simulink model "Lab6"  (R2023a)
settings: Solver=FixedStepDiscrete  StartTime=0.0  StopTime=1000  FixedStep=1/MultiDeviceDAQ_getSampleRate  RelTol=1e-3  EnableMultiTasking=on
InitFcn:
  | clear global handle
  | 
  | clear global userData
  | 
  | tmp_string = gcb;
  | modelname = tmp_string(1:findstr(tmp_string, '/'));
  | method_name = sprintf('%sSignal Processing', modelname);
  | method_val = get_param(method_name,'method');
  | 
  | if exist('P300classifier') ~=1 || (strcmp(method_val, 'Linear Discriminant Analysis') && P300classifier.method ~= 1) || (strcmp(method_val, 'Support Vector Machine') && P300classifier.method ~= 2)
  | try
  | if strcmp(method_val, 'Linear Discriminant Analysis')
  | load lda_rowcolumn_classifier.mat
  | elseif strcmp(method_val, 'Support Vector Machine')
  | load svm_rowcolumn_classifier.mat
  | else
  | global P300classifier
  | P300classifier.method = 0;
  | end
  | catch
  | global P300classifier
  | P300classifier.method = 0;
  | end
  | end
StartFcn:
  | tmp_string = gcb;
  | modelname = tmp_string(1:findstr(tmp_string, '/'));
  | stopsimu_name = sprintf('%sRowCol Character Speller/StopSimu', modelname);
  | set_param(stopsimu_name,'Gain','0');
undefined symbols (not defined in the file): MultiDeviceDAQ_getNumChannels, MultiDeviceDAQ_getSampleRate
libraries: FeatureExtraction x2, Transformation x2, Visualization x2, dspstat3 x1, Preprocessing x1, simulink x1, Classification x1, DataAcquisition x1
settings Model: ModifiedByFormat=g.tec  Creator=circuit  LastModifiedBy=g.tec
settings SolverCC: AlgebraicLoopSolver=TrustRegion
settings DataIOCC: LimitDataPoints=on  SaveFormat=Array  SignalLoggingSaveFormat=ModelDataLogs  ReturnWorkspaceOutputs=off
settings OptimizationCC: ExpressionDepthLimit=2147483647  InitFltsAndDblsToZero=on  LifeSpan=inf
settings DebuggingCC: SaveWithParameterizedLinksMsg=none  UnderspecifiedInitializationDetection=Classic  MergeDetectMultiDrivingBlocksExec=none  SignalResolutionControl=TryResolveAllWithWarning  SolverPrmCheckMsg=warning  MultiTaskDSMMsg=warning  MultiTaskCondExecSysMsg=none  FcnCallInpInsideContextMsg=warning  UnconnectedInputMsg=warning  UnconnectedOutputMsg=warning  UnconnectedLineMsg=warning  FrameProcessingCompatibilityMsg=none  StateNameClashWarn=warning  SFUnexpectedBacktrackingDiag=warning  SFNoUnconditionalDefaultTransitionDiag=warning  SFExecutionAtInitializationDiag=none  ArithmeticOperatorsInVariantConditions=warning
settings HardwareCC: ProdBitPerPointer=32  ProdBitPerSizeT=32  ProdBitPerPtrDiffT=32  ProdLargestAtomicFloat=None  ProdIntDivRoundTo=Undefined  ProdEndianess=Unspecified  ProdWordSize=32  ProdHWDeviceType=32-bit Generic
settings ModelReferenceCC: EnableRefExpFcnMdlSchedulingChecks=on  PropagateSignalLabelsOutOfModel=off
settings SFSimCC: SimUseLocalCustomCode=off  CustomCodeUndefinedFunction=UseInterfaceOnly
settings RTWCC: RTWUseLocalCustomCode=off
settings CodeAppCC: StateflowObjectComments=on
settings GRTTargetCC: TargetFcnLib=ansi_tfl_tmw.mat  TargetLangStandard=C89/C90 (ANSI)  CombineOutputUpdateFcns=off  GRTInterface=on
settings ConfigComp: CovMetricSettings=dw  CovSaveCumulativeToWorkspaceVar=on  CovSaveSingleToWorkspaceVar=on  CovExternalEMLEnable=off

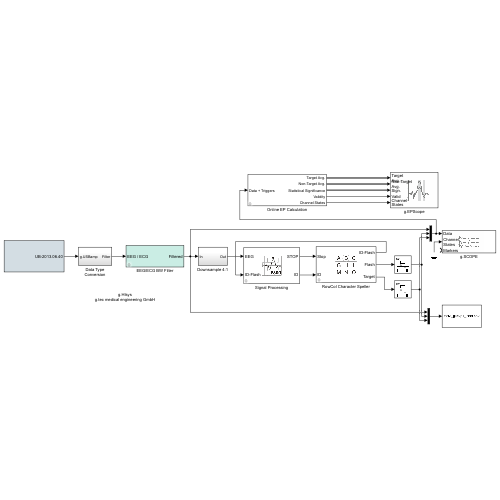
[thumbnail: Simulink's stored preview of the top-level diagram]
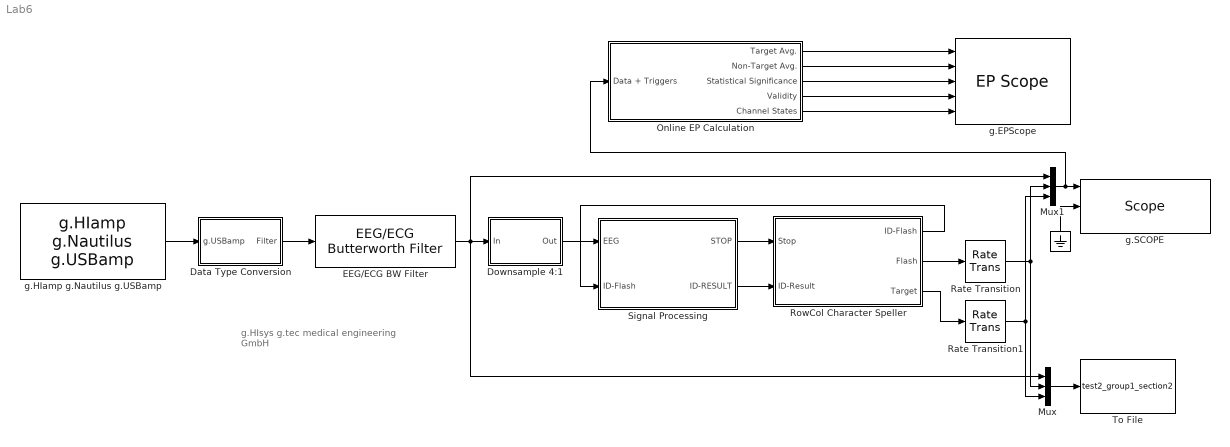
== system Lab6 ==
  note: g.HIsys
      | g.tec medical engineering GmbH
  " " : Ground
  Data Type Conversion : Subsystem
  Downsample 4:1 : Subsystem
  EEG/ECG BW Filter : Preprocessing/EEG//ECG Butterworth Filter  Order=6  LowerFreq=0.1  UpperFreq=30  SampFreq=MultiDeviceDAQ_getSampleRate
      settings: SourceProductName=g.HIsys
  Mux : Mux  Inputs=3
  Mux1 : Mux  Inputs=3
  Online EP Calculation : Subsystem  mask(Online EP Calculation){data_ch_count=MultiDeviceDAQ_getNumChannels, sampletime=1/MultiDeviceDAQ_getSampleRate}
      mask prompts: data_ch_count "Number of data channels:"; sampletime "Sampling time"
      mask help:
      | Calculates the target and non-target average of the incoming data and performs statistical significance analysis of target and non-target frames.
      | The data coming in must contain 'Number of data channel' data channels, trigger IDs and target triggers.
  Rate Transition : RateTransition
  Rate Transition1 : RateTransition
  RowCol Character Speller : Subsystem  mask(Single Character Flash Speller){mode=Copy Spelling, flashtime=100, darktime=75}
      mask prompts: flashtime "Flash time [ms]:"; darktime "Dark time [ms]:"
      mask help: Displays a 36 character matrix. A row or a column of characters is flashing up for a specific time in a random and sequential order. The dark time is the time between the characters.
      mask Help:
      | Displays a 36 character matrix. A row or a column of characters is flashing up for a specific time in a random and sequential order. The dark time is the time between the characters. If the row/column is flashing up the ID-Flash is transmitted for the Signal Processing. Flash contains the ID of every character in the row/column. Target is one if a specific character for the copy spelling mode flashes up. <br><br>
      | 
      | Mode - can be Copy Spelling or Free Spelling<br><br>
      | Flash time [ms] - time that character is shown on screen <br><br>
      | Dark time [ms] - time between the characters
      mask TypeOptions mode: Copy Spelling | Free Spelling
      mask Display:
      | image(imread('speller2.tif'))
      | port_label('output',1,'ID-Flash')
      | port_label('output',2,'Flash')
      | port_label('output',3,'Target')
      | port_label('input',1,'Stop')
      | port_label('input',2,'ID')
  Signal Processing : Subsystem  mask(P300 Signal Processing){windTime=800, runmax=15, channels=8, method=Linear Discriminant Analysis}
      mask prompts: windTime "Buffer length [ms]:"; runmax "Number of flashes:"; channels "Number of channels:"; method "Classification Method:"
      mask help: The block buffers EEG data for each ID-Flash obtained. As soon as M (Number of flashes) characters of each ID are obtained a STOP command is sent and the maximum P300 is calculated and applied on output ID.
      mask Help:
      | P300 Signal Processing block. The block buffers EEG data for each ID-Flash obtained. As soon as M (Number of flashes) characters of each ID are obtained a STOP command is sent. Then the maximum P300 is calculated and the character ID is sent. <br><br>
      | 
      | Buffer length [ms] - enter the EEG data buffer size <br><br>
      | Number of flashes - enter the number each character should flash up <br><br>
      mask TypeOptions method: Linear Discriminant Analysis | Support Vector Machine
      mask Display:
      | image(imread('p3002.tif'))
      | port_label('output', 1, 'STOP')
      | port_label('output', 2, 'ID')
      | port_label('input', 1, 'EEG')
      | port_label('input', 2, 'ID-Flash')
  To File : ToFile  Filename=test2_group1_section2  MatrixName=y  SampleTime=1/MultiDeviceDAQ_getSampleRate
  g.EPScope : Visualization/EP Scope
      settings: SourceProductName=g.HIsys
  g.HIamp g.Nautilus g.USBamp : DataAcquisition/g.HIamp g.Nautilus g.USBamp  cfgUpdated=739906.4436  numDevices=2  deviceSR=[500 250 ]  deviceChannels=[9 4 ]  numSR=[2 ]  SRIndexPerDevice=[1 0 ]
      settings: SourceProductName=g.HIsys
  g.SCOPE : Visualization/Scope
      settings: SourceProductName=g.HIsys
  wires:
  g.HIamp g.Nautilus g.USBamp/1 -> Data Type Conversion/1(g.USBamp)
  Data Type Conversion/1(Filter) -> EEG/ECG BW Filter/1
  EEG/ECG BW Filter/1 -> Mux1/1, Downsample 4:1/1(In), Mux/1
  Signal Processing/1(STOP) -> RowCol Character Speller/1(Stop)
  Signal Processing/2(ID-RESULT) -> RowCol Character Speller/2(ID-Result)
  RowCol Character Speller/1(ID-Flash) -> Signal Processing/2(ID-Flash)
  RowCol Character Speller/2(Flash) -> Rate Transition/1
  RowCol Character Speller/3(Target) -> Rate Transition1/1
  Rate Transition/1 -> Mux1/2, Mux/2
  Rate Transition1/1 -> Mux1/3, Mux/3
  Downsample 4:1/1(Out) -> Signal Processing/1(EEG)
  Mux1/1 -> Online EP Calculation/1(Data + Triggers), g.SCOPE/1
  Mux/1 -> To File/1
  " "/1 -> g.SCOPE/2
  Online EP Calculation/2(Non-Target Avg.) -> g.EPScope/2
  Online EP Calculation/3(Statistical Significance) -> g.EPScope/3
  Online EP Calculation/4(Validity) -> g.EPScope/4
  Online EP Calculation/1(Target Avg.) -> g.EPScope/1
  Online EP Calculation/5(Channel States) -> g.EPScope/5

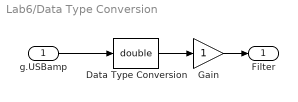
== system Lab6/Data Type Conversion ==
  g.USBamp : Inport  Priority=1
  Data Type Conversion : DataTypeConversion  OutDataTypeStr=double  SaturateOnIntegerOverflow=off  RndMeth=Floor
  Gain : Gain  SaturateOnIntegerOverflow=on  SampleTime=1/MultiDeviceDAQ_getSampleRate  OutDataTypeStr=Inherit: Same as input  ParamDataTypeStr=Inherit: Same as input
  Filter : Outport
  wires:
  Data Type Conversion/1 -> Gain/1
  g.USBamp/1 -> Data Type Conversion/1
  Gain/1 -> Filter/1

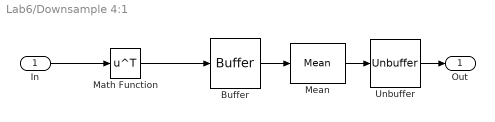
== system Lab6/Downsample 4:1 ==
  In : Inport
  Buffer : Buffer  N=4
  Math Function : Math  Operator=transpose  SignedPower=on
  Mean : dspstat3/Mean  run=off  InputProcessing=Columns as channels (frame based)  reset_popup=None  directionMode=Each column  dimension=1  roiEnable=off  roiType=Rectangles  roiPortion=Entire ROI  roiOutput=Individual statistics for each ROI  roiFlag=off  roundingMode=Floor  overflowMode=off  outputDataTypeStr=Inherit: Same as accumulator  outputMin=[]  outputMax=[]  outputLastDataTypeStr=Inherit: Same as accumulator
  Unbuffer : Unbuffer
  Out : Outport
  wires:
  Buffer/1 -> Mean/1
  Mean/1 -> Unbuffer/1
  In/1 -> Math Function/1
  Unbuffer/1 -> Out/1
  Math Function/1 -> Buffer/1

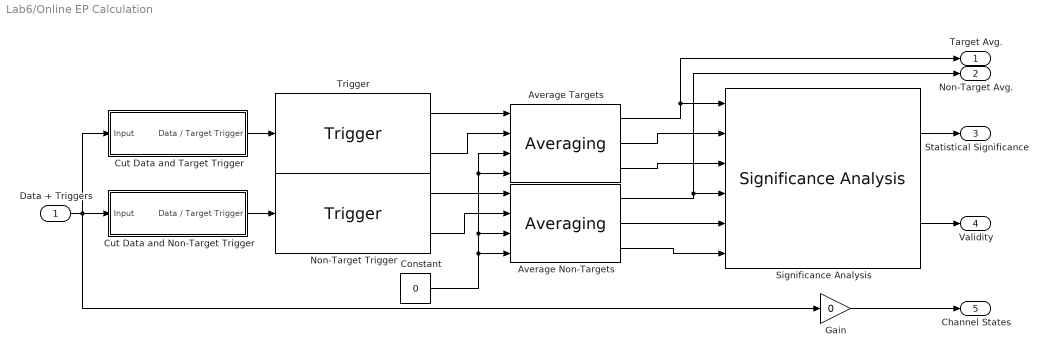
== system Lab6/Online EP Calculation ==
  Data + Triggers : Inport
  Average Non-Targets : FeatureExtraction/Averaging  mode_select=1 - average all data  mode=0  window=3  add_std=on  do_baseline_correction=off  baseline_interval=[0 0]  sampletime=sampletime
      settings: SourceProductName=g.HIsys
  Average Targets : FeatureExtraction/Averaging  mode_select=1 - average all data  mode=0  window=3  add_std=on  do_baseline_correction=off  baseline_interval=[0 0]  sampletime=sampletime
      settings: SourceProductName=g.HIsys
  Constant : Constant  Value=0
  Cut Data and Non-Target Trigger : Subsystem
  Cut Data and Target Trigger : Subsystem
  Gain : Gain  Gain=0
  Non-Target Trigger : Transformation/Trigger  trigchan=9  edge_select=RISING  edge=0  treshold=1  ext_treshold=off  windowsize=0.7  pretrigger=-0.1  sampletime=sampletime  validity_select=STANDARD (global validity flag for all channels)  validity=0  discardTriggerChannels=off
      settings: SourceProductName=g.HIsys
  Significance Analysis : Classification/Significance Analysis  sampletime=sampletime  pValue_select=4 - 0.95  pValue=3  update_mode_select=1 - any Group  update_mode=0
      settings: SourceProductName=g.HIsys
  Trigger : Transformation/Trigger  trigchan=9  edge_select=RISING  edge=0  treshold=1  ext_treshold=off  windowsize=0.7  pretrigger=-0.1  sampletime=sampletime  validity_select=STANDARD (global validity flag for all channels)  validity=0  discardTriggerChannels=off
      settings: SourceProductName=g.HIsys
  Target Avg. : Outport
  Non-Target Avg. : Outport  Port=2
  Statistical Significance : Outport  Port=3
  Validity : Outport  Port=4
  Channel States : Outport  Port=5
  wires:
  Data + Triggers/1 -> Cut Data and Target Trigger/1(Input), Cut Data and Non-Target Trigger/1(Input), Gain/1
  Average Targets/3 -> Significance Analysis/3
  Average Targets/2 -> Significance Analysis/2
  Average Non-Targets/2 -> Significance Analysis/5
  Average Non-Targets/3 -> Significance Analysis/6
  Significance Analysis/2 -> Validity/1
  Trigger/2 -> Average Targets/2
  Trigger/1 -> Average Targets/1
  Non-Target Trigger/1 -> Average Non-Targets/1
  Non-Target Trigger/2 -> Average Non-Targets/2
  Average Targets/1 -> Target Avg./1, Significance Analysis/1
  Average Non-Targets/1 -> Non-Target Avg./1, Significance Analysis/4
  Significance Analysis/1 -> Statistical Significance/1
  Gain/1 -> Channel States/1
  Cut Data and Target Trigger/1(Data / Target Trigger) -> Trigger/1
  Cut Data and Non-Target Trigger/1(Data / Target Trigger) -> Non-Target Trigger/1
  Constant/1 -> Average Non-Targets/4, Average Non-Targets/3, Average Targets/4, Average Targets/3

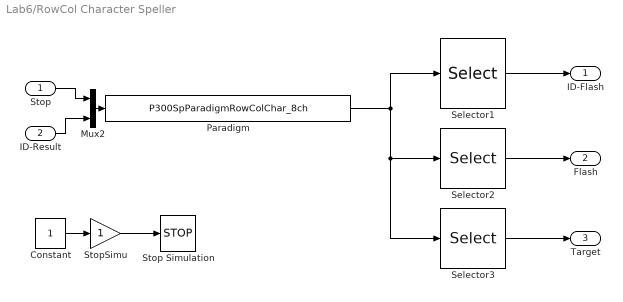
== system Lab6/RowCol Character Speller ==
  Stop : Inport
  ID-Result : Inport  Port=2
  Constant : Constant
  Mux2 : Mux  Inputs=2
  Paradigm : S-Function  FunctionName=P300SpParadigmRowColChar_8ch  Parameters=mode,flashtime,darktime,MultiDeviceDAQ_getSampleRate  SFunctionDeploymentMode=off  EnableBusSupport=off
  Selector1 : Selector  InputPortWidth=9  IndexOptions=Index vector (dialog)  Indices=1:7  OutputSizes=1
  Selector2 : Selector  InputPortWidth=9  IndexOptions=Index vector (dialog)  Indices=[8]  OutputSizes=1
  Selector3 : Selector  InputPortWidth=9  IndexOptions=Index vector (dialog)  Indices=[9]  OutputSizes=1
  Stop Simulation : Stop
  StopSimu : Gain
  ID-Flash : Outport
  Flash : Outport  Port=2
  Target : Outport  Port=3
  wires:
  Stop/1 -> Mux2/1
  ID-Result/1 -> Mux2/2
  Mux2/1 -> Paradigm/1
  Constant/1 -> StopSimu/1
  StopSimu/1 -> Stop Simulation/1
  Paradigm/1 -> Selector1/1, Selector2/1, Selector3/1
  Selector1/1 -> ID-Flash/1
  Selector2/1 -> Flash/1
  Selector3/1 -> Target/1

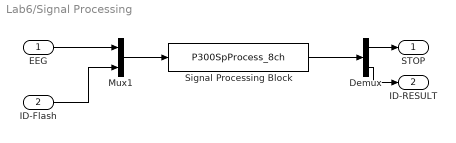
== system Lab6/Signal Processing ==
  EEG : Inport
  ID-Flash : Inport  Port=2
  Demux : Demux  Outputs=2
  Mux1 : Mux  Inputs=2
  Signal Processing Block : S-Function  FunctionName=P300SpProcess_8ch  Parameters=windTime, runmax, channels, method, P300classifier  SFunctionDeploymentMode=off  EnableBusSupport=off
  STOP : Outport
  ID-RESULT : Outport  Port=2
  wires:
  ID-Flash/1 -> Mux1/2
  Demux/1 -> STOP/1
  Demux/2 -> ID-RESULT/1
  Mux1/1 -> Signal Processing Block/1
  Signal Processing Block/1 -> Demux/1
  EEG/1 -> Mux1/1

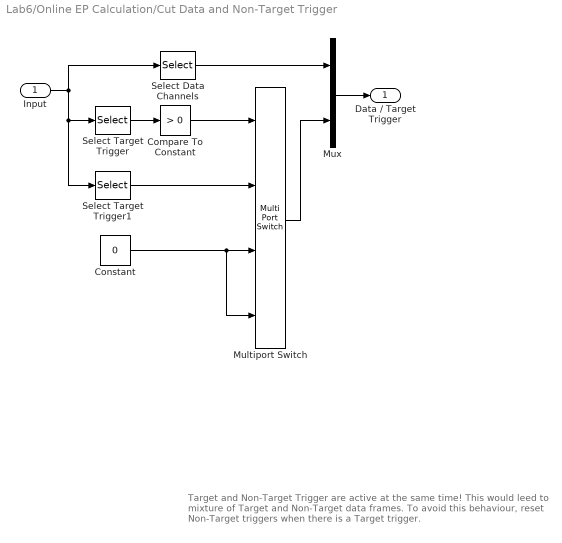
== system Lab6/Online EP Calculation/Cut Data and Non-Target Trigger ==
  note: Target and Non-Target Trigger are active at the same time!
      | This would leed to mixture of Target and Non-Target data frames.
      | To avoid this behaviour, reset Non-Target triggers when there is a Target trigger.
  Input : Inport
  Compare To Constant : simulink/Logic and Bit Operations/Compare To Constant  relop=>  const=0  OutDataTypeStr=uint8
  Constant : Constant  Value=0
  Multiport Switch : MultiPortSwitch  DataPortOrder=Zero-based contiguous  zeroidx=on  SaturateOnIntegerOverflow=off  InputSameDT=off
  Mux : Mux  Inputs=2
  Select Data Channels : Selector  InputPortWidth=data_ch_count + 2  IndexOptions=Index vector (dialog)  Indices=[1:data_ch_count]  OutputSizes=1
  Select Target Trigger : Selector  InputPortWidth=data_ch_count + 2  IndexOptions=Index vector (dialog)  Indices=data_ch_count+2  OutputSizes=1
  Select Target Trigger1 : Selector  InputPortWidth=data_ch_count + 2  IndexOptions=Index vector (dialog)  Indices=data_ch_count+1  OutputSizes=1
  Data / Target Trigger : Outport
  wires:
  Select Data Channels/1 -> Mux/1
  Mux/1 -> Data / Target Trigger/1
  Input/1 -> Select Data Channels/1, Select Target Trigger1/1, Select Target Trigger/1
  Select Target Trigger/1 -> Compare To Constant/1
  Select Target Trigger1/1 -> Multiport Switch/2
  Constant/1 -> Multiport Switch/4, Multiport Switch/3
  Compare To Constant/1 -> Multiport Switch/1
  Multiport Switch/1 -> Mux/2

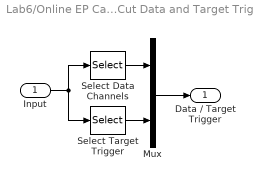
== system Lab6/Online EP Calculation/Cut Data and Target Trigger ==
  Input : Inport
  Mux : Mux  Inputs=2
  Select Data Channels : Selector  InputPortWidth=data_ch_count + 2  IndexOptions=Index vector (dialog)  Indices=[1:data_ch_count]  OutputSizes=1
  Select Target Trigger : Selector  InputPortWidth=data_ch_count + 2  IndexOptions=Index vector (dialog)  Indices=data_ch_count+2  OutputSizes=1
  Data / Target Trigger : Outport
  wires:
  Input/1 -> Select Target Trigger/1, Select Data Channels/1
  Select Target Trigger/1 -> Mux/2
  Mux/1 -> Data / Target Trigger/1
  Select Data Channels/1 -> Mux/1
